simulink model "aerodynamic_model_V1_2_Wrench"  (R2025b)
settings: Solver=ode4  StartTime=0.0  StopTime=0.3  FixedStep=Ts  RelTol=1e-3
InitFcn:
  | % Run initial_main.m first to load Ad,As,Tq_prop,Tq_mass,...
values from neighbouring files (symbols this model uses):
  alpha_du0_v_tail_L = trim_aero_ic.v_tail_L.alpha_du0    [initial_main_V1_1.m]
  alpha_du0_v_tail_R = trim_aero_ic.v_tail_R.alpha_du0    [initial_main_V1_1.m]
  alpha_du0_wing_L = trim_aero_ic.wing_L.alpha_du0    [initial_main_V1_1.m]
  alpha_du0_wing_R = trim_aero_ic.wing_R.alpha_du0    [initial_main_V1_1.m]
  As = sys_sd.A    [initial_main_V1_1.m]
  BladePitch_deg = 34    [initial_main_V1_1.m]
  Bs = sys_sd.B    [initial_main_V1_1.m]
  Cs = sys_sd.C    [initial_main_V1_1.m]
  ctrl_delta_lim_deg = strips.delta_lim_deg    [initial_main_V1_1.m]
  ctrl_map_aileron_L = aero.wing_L.map_aileron(:)    [initial_main_V1_1.m]
  ctrl_map_aileron_R = aero.wing_R.map_aileron(:)    [initial_main_V1_1.m]
  ctrl_map_tail_L = aero.v_tail_L.map_tail(:)    [initial_main_V1_1.m]
  ctrl_map_tail_R = aero.v_tail_R.map_tail(:)    [initial_main_V1_1.m]
  Ds = sys_sd.D    [initial_main_V1_1.m]
  I_cg_b = R_sb * I_cg_m * R_sb.'    [aeroelastic.m]    (also in initial_main_V1_1.m = grav.I_cg_b)
  I_cg_b_inv = R_sb * I_cg_m_inv * R_sb.'    [aeroelastic.m]    (also in initial_main_V1_1.m = grav.I_cg_b_inv)
  m_node = zeros(n_id, 1)    [aeroelastic.m]    (also in generate_pullup_load_cloud.m = evalin('base', 'm_node(:)'); initial_main_V1_1.m = nodal.m_node)
  m_total_kg = evalin('base', 'm_total_kg')    [generate_pullup_load_cloud.m]    (also in initial_main_V1_1.m = grav.m_total_kg)
  n_modes = size(Phi, 2)    [aeroelastic.m]    (also in initial_main_V1_1.m = n_rigid + n_elastic)
  ones_1_tail = ones(1, size(r_cg2ac_b_v_tail_L, 2))    [initial_main_V1_1.m]
  ones_1_wing = ones(1, size(r_cg2ac_b_wing_L, 2))    [initial_main_V1_1.m]
  Phi = evalin('base', 'Phi')    [generate_pullup_load_cloud.m]    (also in initial_main_V1_1.m = strips.Phi)
  polar_alpha_deg = polar.alpha_deg(:).'    [initial_main_V1_1.m]
  polar_CD = polar.CD(:).'    [initial_main_V1_1.m]
  polar_CDp = polar.CDp(:).'    [initial_main_V1_1.m]
  polar_CL = polar.CL(:).'    [initial_main_V1_1.m]
  polar_CM = polar.CM(:).'    [initial_main_V1_1.m]
  r_cg2ac_b_v_tail_L = R_sb * aero.v_tail_L.r_ac_s    [initial_main_V1_1.m]
  r_cg2ac_b_v_tail_R = R_sb * aero.v_tail_R.r_ac_s    [initial_main_V1_1.m]
  r_cg2ac_b_wing_L = R_sb * aero.wing_L.r_ac_s    [initial_main_V1_1.m]
  r_cg2ac_b_wing_R = R_sb * aero.wing_R.r_ac_s    [initial_main_V1_1.m]
  r_cg2kink_b = eng.r_cg2kink_b    [initial_main_V1_1.m]
  r_cg2node_b = aeroelastic.node_arms(nodes, 'R_sb', R_sb).r_cg2node_b    [initial_main_V1_1.m]
  surface_nodes = aeroelastic.surface_load_nodes(nodes)    [initial_main_V1_1.m]
  T_aero2W = aeroelastic.wing_aileron_to_W(strips).T    [initial_main_V1_1.m]
  T_prop2W = load_maps.T_prop2W    [initial_main_V1_1.m]
  Tq_mass = load_maps.Tq_mass    [initial_main_V1_1.m]
  trim_Attitude_rad0 = trim_default.Attitude_rad0    [initial_main_V1_1.m]
  trim_Omega_b0 = trim_default.Omega_b0    [initial_main_V1_1.m]
  trim_Position0 = trim_default.Position0    [initial_main_V1_1.m]
  trim_Velocity_b0 = trim_default.Velocity_b0    [initial_main_V1_1.m]
  Ts = 0.001    [initial_main_V1_1.m]
  U = 55    [initial_main_V1_1.m]
  v_tail_cant_rad = deg2rad(v_tail_cant_deg)    [initial_main_V1_1.m]
  W_mass_g = grav.W_mass    [initial_main_V1_1.m]
  x0_structure = trim_default.x0_structure    [initial_main_V1_1.m]
  x0_wagner_v_tail_L = trim_aero_ic.v_tail_L.x0_wagner    [initial_main_V1_1.m]
  x0_wagner_v_tail_R = trim_aero_ic.v_tail_R.x0_wagner    [initial_main_V1_1.m]
  x0_wagner_wing_L = trim_aero_ic.wing_L.x0_wagner    [initial_main_V1_1.m]
  x0_wagner_wing_R = trim_aero_ic.wing_R.x0_wagner    [initial_main_V1_1.m]
undefined symbols (not defined in the file or in its folder): Ad_v_tail_L, Ad_v_tail_R, Ad_wing_L, Ad_wing_R, Bd_v_tail_L, Bd_v_tail_R, Bd_wing_L, Bd_wing_R, c_over_2U_v_tail_L, c_over_2U_v_tail_R, c_over_2U_wing_L, c_over_2U_wing_R, Cd_v_tail_L, Cd_v_tail_R, Cd_wing_L, Cd_wing_R, Dd_v_tail_L, Dd_v_tail_R, Dd_wing_L, Dd_wing_R, G_du_v_tail_L, G_du_v_tail_R, G_du_wing_L, G_du_wing_R, polar_aileron_alpha_deg, polar_aileron_dCD, polar_aileron_dCL, polar_aileron_dCM, polar_aileron_delta_deg, polar_ruddervator_alpha_deg, polar_ruddervator_dCD, polar_ruddervator_dCL, polar_ruddervator_dCM, polar_ruddervator_delta_deg, qS_strip_v_tail_L, qS_strip_v_tail_R, qS_strip_wing_L, qS_strip_wing_R, qSc_strip_v_tail_L, qSc_strip_v_tail_R, qSc_strip_wing_L, qSc_strip_wing_R, T_m2b_v_tail_L, T_m2b_v_tail_R, T_m2b_wing_L, T_m2b_wing_R, T_m2h_v_tail_L, T_m2h_v_tail_R, T_m2h_wing_L, T_m2h_wing_R, Tq_CM_v_tail_L, Tq_CM_v_tail_R, Tq_CM_wing_L, Tq_CM_wing_R, Tq_D_v_tail_L, Tq_D_v_tail_R, Tq_D_wing_L, Tq_D_wing_R, Tq_v_tail_L, Tq_v_tail_R ... (+2)
libraries: Prop_gryo x12, matrix_library x2
(part 5 of 6)

== system aerodynamic_model_V1_2_Wrench/Load Estimator/Engine_station1/Subsystem6 ==
  Wb_total : Inport
  r_cg_up : Inport  Port=2
  tilt_deg : Inport  Port=3
  Bus Creator : BusCreator  Inputs=6
  Bus Creator1 : BusCreator  Inputs=6
  Bus Creator2 : BusCreator  Inputs=6
  Bus Creator4 : BusCreator  Inputs=3
  Constant : Constant  Value=r_cg2node_b(:,61)
  Constant1 : Constant  Value=r_cg2node_b(:,60)
  Constant2 : Constant  Value=0
  Constant3 : Constant  Value=r_cg2node_b(:,28)
  Constant4 : Constant  Value=[0 0 0]/180*pi
  Constant5 : Constant  Value=[7 0 0]/180*pi
  Constant6 : Constant  Value=-7
  Demux{1..6} (6 alike) : Demux  Outputs=3
  Gain : Gain  Gain=pi/180
  MATLAB Function1 : MATLAB Function  TreatAsAtomicUnit=on
  MATLAB Function2 : MATLAB Function  TreatAsAtomicUnit=on
  MATLAB Function3 : MATLAB Function  TreatAsAtomicUnit=on
  Mux : Mux  Inputs=3
  Product{1..4,6..7} (6 alike) : Product  Multiplication=Matrix(*)
  Rotation Angles to Direction Cosine Matrix : Angle2Dcm  rotationOrder=XYZ
      settings: AttributesFormatString=Rotation Order: %<rotationOrder>
  Rotation Angles to Direction Cosine Matrix1 : Angle2Dcm  rotationOrder=XYZ
      settings: AttributesFormatString=Rotation Order: %<rotationOrder>
  Rotation Angles to Direction Cosine Matrix2 : Angle2Dcm  rotationOrder=XYZ
      settings: AttributesFormatString=Rotation Order: %<rotationOrder>
  Selector1 : Selector  NumberOfDimensions=2  InputPortWidth=3  IndexOptions=Select all,Index vector (dialog)  Indices=[1:6],[61]  OutputSizes=1,1
  Selector10 : Selector  NumberOfDimensions=2  InputPortWidth=3  IndexOptions=Index vector (dialog),Select all  Indices=[4:6],[surface_nodes.wing_R.node_id]  OutputSizes=1,1
  Selector11 : Selector  NumberOfDimensions=2  InputPortWidth=3  IndexOptions=Index vector (dialog),Select all  Indices=[4:6],[surface_nodes.wing_R.node_id]  OutputSizes=1,1
  Selector12 : Selector  NumberOfDimensions=2  InputPortWidth=3  IndexOptions=Index vector (dialog),Select all  Indices=[1:3],[surface_nodes.wing_R.node_id]  OutputSizes=1,1
  Selector13 : Selector  NumberOfDimensions=2  InputPortWidth=3  IndexOptions=Index vector (dialog),Select all  Indices=[4:6],[surface_nodes.wing_R.node_id]  OutputSizes=1,1
  Selector14 : Selector  NumberOfDimensions=2  InputPortWidth=3  IndexOptions=Index vector (dialog),Select all  Indices=[1:3],[surface_nodes.wing_R.node_id]  OutputSizes=1,1
  Selector2 : Selector  NumberOfDimensions=2  InputPortWidth=3  IndexOptions=Select all,Index vector (dialog)  Indices=[1:6],[60 61]  OutputSizes=1,1
  Selector3 : Selector  NumberOfDimensions=2  InputPortWidth=3  IndexOptions=Select all,Index vector (dialog)  Indices=[1:6],[61]  OutputSizes=1,1
  Selector4 : Selector  NumberOfDimensions=2  InputPortWidth=3  IndexOptions=Select all,Index vector (dialog)  Indices=[1:6],[60 61]  OutputSizes=1,1
  Selector5 : Selector  NumberOfDimensions=2  InputPortWidth=3  IndexOptions=Select all,Index vector (dialog)  Indices=[1:6],[59:61]  OutputSizes=1,1
  Selector6 : Selector  NumberOfDimensions=2  InputPortWidth=3  IndexOptions=Select all,Index vector (dialog)  Indices=[1:6],[59:61]  OutputSizes=1,1
  Selector9 : Selector  NumberOfDimensions=2  InputPortWidth=3  IndexOptions=Index vector (dialog),Select all  Indices=[1:3],[surface_nodes.wing_R.node_id]  OutputSizes=1,1
  Out1 : Outport
  wires:
  Demux3/3 -> Bus Creator2/3  "shear_forcez"
  Selector4/1 -> MATLAB Function2/3(r)
  MATLAB Function3/2(M_b) -> Product4/2
  MATLAB Function1/2(M_b) -> Product7/2
  Demux1/2 -> Bus Creator1/2  "shear_forcey"
  Demux6/3 -> Bus Creator2/6  "Bending_momenty"
  MATLAB Function1/1(F_b) -> Product6/2
  Selector6/1 -> MATLAB Function3/3(r)
  Demux1/3 -> Bus Creator1/3  "shear_forcez"
  Demux5/2 -> Bus Creator/5  "Bending_momentx"
  Selector2/1 -> Selector11/1, Selector12/1
  Demux4/2 -> Bus Creator/2  "shear_forcey"
  Selector12/1 -> MATLAB Function2/1(F)
  Bus Creator1/1 -> Bus Creator4/2
  Demux5/3 -> Bus Creator/6  "Bending_momenty"
  Selector5/1 -> Selector13/1, Selector14/1
  Constant1/1 -> MATLAB Function2/4(p)
  Demux5/1 -> Bus Creator/4  "Torision_moment"
  Constant2/1 -> Mux/3
  Gain/1 -> Rotation Angles to Direction Cosine Matrix/1
  Bus Creator2/1 -> Bus Creator4/3
  Product3/1 -> Demux3/1
  Demux1/1 -> Bus Creator1/1  "Axial_Force"
  Selector9/1 -> MATLAB Function1/1(F)
  Product7/1 -> Demux5/1
  Bus Creator/1 -> Bus Creator4/1
  Demux4/1 -> Bus Creator/1  "Axial_Force"
  Wb_total/1 -> Selector2/1, Selector5/1, Selector1/1
  Demux2/1 -> Bus Creator1/4  "Torision_moment"
  Rotation Angles to Direction Cosine Matrix2/1 -> Product4/1, Product3/1
  Constant6/1 -> Mux/1
  Mux/1 -> Gain/1
  Product6/1 -> Demux4/1
  Demux3/1 -> Bus Creator2/1  "Axial_Force"
  Selector11/1 -> MATLAB Function2/2(M)
  Demux6/1 -> Bus Creator2/4  "Torision_moment"
  Demux2/3 -> Bus Creator1/6  "Bending_momenty"
  MATLAB Function2/1(F_b) -> Product1/2
  Rotation Angles to Direction Cosine Matrix1/1 -> Product1/1, Product2/1
  Demux4/3 -> Bus Creator/3  "shear_forcez"
  Constant3/1 -> MATLAB Function3/4(p)
  Product1/1 -> Demux1/1
  Product2/1 -> Demux2/1
  Constant5/1 -> Rotation Angles to Direction Cosine Matrix1/1
  MATLAB Function2/2(M_b) -> Product2/2
  Bus Creator4/1 -> Out1/1
  r_cg_up/1 -> Selector6/1, Selector4/1, Selector3/1
  Selector1/1 -> Selector10/1, Selector9/1
  MATLAB Function3/1(F_b) -> Product3/2
  tilt_deg/1 -> Mux/2
  Selector10/1 -> MATLAB Function1/2(M)
  Rotation Angles to Direction Cosine Matrix/1 -> Product7/1, Product6/1
  Selector13/1 -> MATLAB Function3/2(M)
  Constant4/1 -> Rotation Angles to Direction Cosine Matrix2/1
  Selector14/1 -> MATLAB Function3/1(F)
  Demux2/2 -> Bus Creator1/5  "Bending_momentx"
  Demux3/2 -> Bus Creator2/2  "shear_forcey"
  Selector3/1 -> MATLAB Function1/3(r)
  Constant/1 -> MATLAB Function1/4(p)
  Demux6/2 -> Bus Creator2/5  "Bending_momentx"
  Product4/1 -> Demux6/1

== system aerodynamic_model_V1_2_Wrench/Load Estimator/Engine_station1/Subsystem7 ==
  In1 : Inport
  r_cg_up : Inport  Port=2
  Bus Creator : BusCreator  Inputs=6
  Bus Creator1 : BusCreator  Inputs=6
  Bus Creator2 : BusCreator  Inputs=6
  Bus Creator4 : BusCreator  Inputs=3
  Constant : Constant  Value=r_cg2node_b(:,67)
  Constant1 : Constant  Value=r_cg2node_b(:,66)
  Constant2 : Constant  Value=0
  Constant3 : Constant  Value=r_cg2node_b(:,46)
  Constant4 : Constant  Value=[0 0 0]/180*pi
  Constant5 : Constant  Value=[-7 0 0]/180*pi
  Constant6 : Constant  Value=-7
  Constant7 : Constant  Value=90
  Demux{1..6} (6 alike) : Demux  Outputs=3
  Gain : Gain  Gain=pi/180
  MATLAB Function1 : MATLAB Function  TreatAsAtomicUnit=on
  MATLAB Function2 : MATLAB Function  TreatAsAtomicUnit=on
  MATLAB Function3 : MATLAB Function  TreatAsAtomicUnit=on
  Mux : Mux  Inputs=3
  Product{1..4,6..7} (6 alike) : Product  Multiplication=Matrix(*)
  Rotation Angles to Direction Cosine Matrix : Angle2Dcm  rotationOrder=XYZ
      settings: AttributesFormatString=Rotation Order: %<rotationOrder>
  Rotation Angles to Direction Cosine Matrix1 : Angle2Dcm  rotationOrder=XYZ
      settings: AttributesFormatString=Rotation Order: %<rotationOrder>
  Rotation Angles to Direction Cosine Matrix2 : Angle2Dcm  rotationOrder=XYZ
      settings: AttributesFormatString=Rotation Order: %<rotationOrder>
  Selector1 : Selector  NumberOfDimensions=2  InputPortWidth=3  IndexOptions=Select all,Index vector (dialog)  Indices=[1:6],[67]  OutputSizes=1,1
  Selector10 : Selector  NumberOfDimensions=2  InputPortWidth=3  IndexOptions=Index vector (dialog),Select all  Indices=[4:6],[surface_nodes.wing_R.node_id]  OutputSizes=1,1
  Selector11 : Selector  NumberOfDimensions=2  InputPortWidth=3  IndexOptions=Index vector (dialog),Select all  Indices=[4:6],[surface_nodes.wing_R.node_id]  OutputSizes=1,1
  Selector12 : Selector  NumberOfDimensions=2  InputPortWidth=3  IndexOptions=Index vector (dialog),Select all  Indices=[1:3],[surface_nodes.wing_R.node_id]  OutputSizes=1,1
  Selector13 : Selector  NumberOfDimensions=2  InputPortWidth=3  IndexOptions=Index vector (dialog),Select all  Indices=[4:6],[surface_nodes.wing_R.node_id]  OutputSizes=1,1
  Selector14 : Selector  NumberOfDimensions=2  InputPortWidth=3  IndexOptions=Index vector (dialog),Select all  Indices=[1:3],[surface_nodes.wing_R.node_id]  OutputSizes=1,1
  Selector2 : Selector  NumberOfDimensions=2  InputPortWidth=3  IndexOptions=Select all,Index vector (dialog)  Indices=[1:6],[66 67]  OutputSizes=1,1
  Selector3 : Selector  NumberOfDimensions=2  InputPortWidth=3  IndexOptions=Select all,Index vector (dialog)  Indices=[1:6],[67]  OutputSizes=1,1
  Selector4 : Selector  NumberOfDimensions=2  InputPortWidth=3  IndexOptions=Select all,Index vector (dialog)  Indices=[1:6],[66 67]  OutputSizes=1,1
  Selector5 : Selector  NumberOfDimensions=2  InputPortWidth=3  IndexOptions=Select all,Index vector (dialog)  Indices=[1:6],[65:67]  OutputSizes=1,1
  Selector6 : Selector  NumberOfDimensions=2  InputPortWidth=3  IndexOptions=Select all,Index vector (dialog)  Indices=[1:6],[65:67]  OutputSizes=1,1
  Selector9 : Selector  NumberOfDimensions=2  InputPortWidth=3  IndexOptions=Index vector (dialog),Select all  Indices=[1:3],[surface_nodes.wing_R.node_id]  OutputSizes=1,1
  Out1 : Outport
  wires:
  Product4/1 -> Demux6/1
  Demux6/2 -> Bus Creator2/5  "Bending_momentx"
  Constant/1 -> MATLAB Function1/4(p)
  Selector3/1 -> MATLAB Function1/3(r)
  Demux3/2 -> Bus Creator2/2  "shear_forcey"
  Demux2/2 -> Bus Creator1/5  "Bending_momentx"
  Selector14/1 -> MATLAB Function3/1(F)
  Constant4/1 -> Rotation Angles to Direction Cosine Matrix2/1
  Selector13/1 -> MATLAB Function3/2(M)
  Rotation Angles to Direction Cosine Matrix/1 -> Product6/1, Product7/1
  Selector10/1 -> MATLAB Function1/2(M)
  Constant7/1 -> Mux/2
  MATLAB Function3/1(F_b) -> Product3/2
  Selector1/1 -> Selector9/1, Selector10/1
  r_cg_up/1 -> Selector3/1, Selector4/1, Selector6/1
  Bus Creator4/1 -> Out1/1
  MATLAB Function2/2(M_b) -> Product2/2
  Constant5/1 -> Rotation Angles to Direction Cosine Matrix1/1
  Product2/1 -> Demux2/1
  Product1/1 -> Demux1/1
  Constant3/1 -> MATLAB Function3/4(p)
  Demux4/3 -> Bus Creator/3  "shear_forcez"
  Rotation Angles to Direction Cosine Matrix1/1 -> Product2/1, Product1/1
  MATLAB Function2/1(F_b) -> Product1/2
  Demux2/3 -> Bus Creator1/6  "Bending_momenty"
  Demux6/1 -> Bus Creator2/4  "Torision_moment"
  Selector11/1 -> MATLAB Function2/2(M)
  Demux3/1 -> Bus Creator2/1  "Axial_Force"
  Product6/1 -> Demux4/1
  Mux/1 -> Gain/1
  Constant6/1 -> Mux/1
  Rotation Angles to Direction Cosine Matrix2/1 -> Product3/1, Product4/1
  Demux2/1 -> Bus Creator1/4  "Torision_moment"
  In1/1 -> Selector2/1, Selector5/1, Selector1/1
  Demux4/1 -> Bus Creator/1  "Axial_Force"
  Bus Creator/1 -> Bus Creator4/1
  Product7/1 -> Demux5/1
  Selector9/1 -> MATLAB Function1/1(F)
  Demux1/1 -> Bus Creator1/1  "Axial_Force"
  Product3/1 -> Demux3/1
  Bus Creator2/1 -> Bus Creator4/3
  Gain/1 -> Rotation Angles to Direction Cosine Matrix/1
  Constant2/1 -> Mux/3
  Demux5/1 -> Bus Creator/4  "Torision_moment"
  Constant1/1 -> MATLAB Function2/4(p)
  Selector5/1 -> Selector14/1, Selector13/1
  Demux5/3 -> Bus Creator/6  "Bending_momenty"
  Bus Creator1/1 -> Bus Creator4/2
  Selector12/1 -> MATLAB Function2/1(F)
  Demux4/2 -> Bus Creator/2  "shear_forcey"
  Selector2/1 -> Selector12/1, Selector11/1
  Demux5/2 -> Bus Creator/5  "Bending_momentx"
  Demux1/3 -> Bus Creator1/3  "shear_forcez"
  Selector6/1 -> MATLAB Function3/3(r)
  MATLAB Function1/1(F_b) -> Product6/2
  Demux6/3 -> Bus Creator2/6  "Bending_momenty"
  Demux1/2 -> Bus Creator1/2  "shear_forcey"
  MATLAB Function1/2(M_b) -> Product7/2
  MATLAB Function3/2(M_b) -> Product4/2
  Selector4/1 -> MATLAB Function2/3(r)
  Demux3/3 -> Bus Creator2/3  "shear_forcez"

== matlab function aerodynamic_model_V1_2_Wrench/Strip Aerodynamics/Local_Alphas/MATLAB Function1 ==
  data: V input; alpha output; beta output
function [alpha, beta] = fcn(V)
[alpha, beta] = strip_aero_angles(V);
end

== matlab function aerodynamic_model_V1_2_Wrench/Strip Aerodynamics/Local_Alphas/MATLAB Function2 ==
  data: V input; alpha output; beta output
function [alpha, beta] = fcn(V)
[alpha, beta] = strip_aero_angles(V);
end

== matlab function aerodynamic_model_V1_2_Wrench/Strip Aerodynamics/Local_Alphas/MATLAB Function4 ==
  data: V input; alpha output; beta output
function [alpha, beta] = fcn(V)
[alpha, beta] = strip_aero_angles(V);
end

== matlab function aerodynamic_model_V1_2_Wrench/Strip Aerodynamics/Local_Alphas/MATLAB Function ==
  data: omega input; Omega_skew output
function Omega_skew = fcn(omega)
p=omega(1);
q=omega(2);
r=omega(3);

Omega_skew =  [0 -r q;r 0 -p;-q p 0];

== matlab function aerodynamic_model_V1_2_Wrench/Load Estimator/Structural_Station_Section/MATLAB Function3 ==
  data: F input; F_b output; M input; r input; M_b output; p input
function [F_b, M_b] = wrench_to_cg(F, M, r,p) %#codegen
%WRENCH_TO_CG  节点力/力矩合到质心
%
%  [F_cg, M_cg] = wrench_to_cg(F, M, r)
%
%  F, M, r  3×n  每列一个节点，必须同一坐标系
%            r 用 r_cg2node_m（结构）或 r_cg2node_b（机体）
%  F_cg     3×1  Σ F
%  M_cg     3×1  Σ (r × F + M)
%
%  不要把 6 维扳手整段叉乘。力只求和；力矩才是 r×F 再加节点力矩。
n=size(r,2);
for i=1:n
    r(:,i)=r(:,i)-p;
end
    F_b = sum(F, 2);
    M_b = sum(cross3n(r, F) + M, 2);
end

== matlab function aerodynamic_model_V1_2_Wrench/Flexible Aircraft Dynamics/MATLAB Function2 ==
  data: F input; F_cg output; M input; r input; M_cg output
function [F_cg, M_cg] = wrench_to_cg(F, M, r) %#codegen
%WRENCH_TO_CG  节点力/力矩合到质心
%
%  [F_cg, M_cg] = wrench_to_cg(F, M, r)
%
%  F, M, r  3×n  每列一个节点，必须同一坐标系
%            r 用 r_cg2node_m（结构）或 r_cg2node_b（机体）
%  F_cg     3×1  Σ F
%  M_cg     3×1  Σ (r × F + M)
%
%  不要把 6 维扳手整段叉乘。力只求和；力矩才是 r×F 再加节点力矩。

    F_cg = sum(F, 2);
    M_cg = sum(cross3n(r, F) + M, 2);
end

== matlab function aerodynamic_model_V1_2_Wrench/Load Estimator/MATLAB Function2 ==
  data: V_b input; Acc_b input; a_node output; Omega_b input; rate_b input; r input; m input; F_inertia output; a_cg_up input
function [a_node, F_inertia] = rigid_node_inertia( ...
    V_b, Acc_b, Omega_b, rate_b, r, m, a_cg_up) %#codegen
%RIGID_NODE_INERTIA
% 计算刚体运动条件下各节点的绝对加速度和惯性力
%
% 输入：
%   V_b      3×1   质心速度 [u;v;w]，机体系
%   Acc_b    3×1   速度分量导数 [du/dt;dv/dt;dw/dt]
%   Omega_b  3×1   刚体角速度 [p;q;r]
%   rate_b   3×1   刚体角加速度 [dp/dt;dq/dt;dr/dt]
%   r        3×N   CG到各节点的位置矢量
%   m        N×1   各节点质量
%
% 输出：
%   a_node      3×N  各节点绝对加速度
%   F_inertia   3×N  各节点惯性力
%
% 惯性力采用达朗贝尔形式：
%
%   F_inertia_i = -m_i * a_i
%
% 要求：
%   size(r,2) == length(m)

    % 质心绝对加速度
    % 若 Acc_b 已经是绝对加速度，则这里应直接写：
    % a_cg = Acc_b;
    a_cg = Acc_b + cross(Omega_b, V_b);

    % 节点数量
    n = size(r, 2);

    % 预分配
    a_node    = a_cg_up;
    F_inertia = zeros(6, n);

    % 各节点刚体惯性载荷
    for i = 1:n

        ri = r(:,i);

        % 节点绝对加速度
        a_node(:,i) = a_node(:,i)+ a_cg ...
            + cross(rate_b, ri) ...
            + cross(Omega_b, cross(Omega_b, ri));

        % 节点惯性力
        F_inertia(1:3,i) = -m(i) * a_node(:,i);

    end

end

== matlab function aerodynamic_model_V1_2_Wrench/Flexible Aircraft Dynamics/MATLAB Function3 ==
  data: p input; phi_dot output; q input; r input; phi input; theta input; theta_dot output; psi_dot output
function [phi_dot, theta_dot, psi_dot] = euler_kinematics(p, q, r, phi, theta)
    % 输入：
    %   p, q, r  - 体轴角速度 (rad/s)
    %   phi      - 滚转角 (rad)
    %   theta    - 俯仰角 (rad)
    % 输出：
    %   phi_dot, theta_dot, psi_dot - 欧拉角变化率 (rad/s)
    
    % 保护：防止 theta = ±90° 时除零（万向节锁）
    cos_theta = cos(theta);
    if abs(cos_theta) < 1e-6
        cos_theta = sign(cos_theta) * 1e-6;  % 保留符号，避免符号跳变
    end
    
    tan_theta = sin(theta) / cos_theta;
    
    % 运动学矩阵
    phi_dot   = p + q * sin(phi) * tan_theta + r * cos(phi) * tan_theta;
    theta_dot = q * cos(phi) - r * sin(phi);
    psi_dot   = (q * sin(phi) + r * cos(phi)) / cos_theta;
end

== matlab function aerodynamic_model_V1_2_Wrench/Load Estimator/Engine_station/Subsystem/MATLAB Function1 ==
  data: F input; F_b output; M input; r input; M_b output; p input
function [F_b, M_b] = wrench_to_cg(F, M, r,p) %#codegen
%WRENCH_TO_CG  节点力/力矩合到质心
%
%  [F_cg, M_cg] = wrench_to_cg(F, M, r)
%
%  F, M, r  3×n  每列一个节点，必须同一坐标系
%            r 用 r_cg2node_m（结构）或 r_cg2node_b（机体）
%  F_cg     3×1  Σ F
%  M_cg     3×1  Σ (r × F + M)
%
%  不要把 6 维扳手整段叉乘。力只求和；力矩才是 r×F 再加节点力矩。
n=size(r,2);
for i=1:n
    r(:,i)=r(:,i)-p;
end
    F_b = sum(F, 2);
    M_b = sum(cross3n(r, F) + M, 2);
end

== matlab function aerodynamic_model_V1_2_Wrench/Load Estimator/Engine_station/Subsystem/MATLAB Function2 ==
  data: F input; F_b output; M input; r input; M_b output; p input
function [F_b, M_b] = wrench_to_cg(F, M, r,p) %#codegen
%WRENCH_TO_CG  节点力/力矩合到质心
%
%  [F_cg, M_cg] = wrench_to_cg(F, M, r)
%
%  F, M, r  3×n  每列一个节点，必须同一坐标系
%            r 用 r_cg2node_m（结构）或 r_cg2node_b（机体）
%  F_cg     3×1  Σ F
%  M_cg     3×1  Σ (r × F + M)
%
%  不要把 6 维扳手整段叉乘。力只求和；力矩才是 r×F 再加节点力矩。
n=size(r,2);
for i=1:n
    r(:,i)=r(:,i)-p;
end
    F_b = sum(F, 2);
    M_b = sum(cross3n(r, F) + M, 2);
end

== matlab function aerodynamic_model_V1_2_Wrench/Load Estimator/Engine_station/Subsystem/MATLAB Function3 ==
  data: F input; F_b output; M input; r input; M_b output; p input
function [F_b, M_b] = wrench_to_cg(F, M, r,p) %#codegen
%WRENCH_TO_CG  节点力/力矩合到质心
%
%  [F_cg, M_cg] = wrench_to_cg(F, M, r)
%
%  F, M, r  3×n  每列一个节点，必须同一坐标系
%            r 用 r_cg2node_m（结构）或 r_cg2node_b（机体）
%  F_cg     3×1  Σ F
%  M_cg     3×1  Σ (r × F + M)
%
%  不要把 6 维扳手整段叉乘。力只求和；力矩才是 r×F 再加节点力矩。
n=size(r,2);
for i=1:n
    r(:,i)=r(:,i)-p;
end
    F_b = sum(F, 2);
    M_b = sum(cross3n(r, F) + M, 2);
end

== matlab function aerodynamic_model_V1_2_Wrench/Load Estimator/Engine_station/Subsystem1/MATLAB Function1 ==
  data: F input; F_b output; M input; r input; M_b output; p input
function [F_b, M_b] = wrench_to_cg(F, M, r,p) %#codegen
%WRENCH_TO_CG  节点力/力矩合到质心
%
%  [F_cg, M_cg] = wrench_to_cg(F, M, r)
%
%  F, M, r  3×n  每列一个节点，必须同一坐标系
%            r 用 r_cg2node_m（结构）或 r_cg2node_b（机体）
%  F_cg     3×1  Σ F
%  M_cg     3×1  Σ (r × F + M)
%
%  不要把 6 维扳手整段叉乘。力只求和；力矩才是 r×F 再加节点力矩。
n=size(r,2);
for i=1:n
    r(:,i)=r(:,i)-p;
end
    F_b = sum(F, 2);
    M_b = sum(cross3n(r, F) + M, 2);
end

== matlab function aerodynamic_model_V1_2_Wrench/Load Estimator/Engine_station/Subsystem1/MATLAB Function2 ==
  data: F input; F_b output; M input; r input; M_b output; p input
function [F_b, M_b] = wrench_to_cg(F, M, r,p) %#codegen
%WRENCH_TO_CG  节点力/力矩合到质心
%
%  [F_cg, M_cg] = wrench_to_cg(F, M, r)
%
%  F, M, r  3×n  每列一个节点，必须同一坐标系
%            r 用 r_cg2node_m（结构）或 r_cg2node_b（机体）
%  F_cg     3×1  Σ F
%  M_cg     3×1  Σ (r × F + M)
%
%  不要把 6 维扳手整段叉乘。力只求和；力矩才是 r×F 再加节点力矩。
n=size(r,2);
for i=1:n
    r(:,i)=r(:,i)-p;
end
    F_b = sum(F, 2);
    M_b = sum(cross3n(r, F) + M, 2);
end

== matlab function aerodynamic_model_V1_2_Wrench/Load Estimator/Engine_station/Subsystem1/MATLAB Function3 ==
  data: F input; F_b output; M input; r input; M_b output; p input
function [F_b, M_b] = wrench_to_cg(F, M, r,p) %#codegen
%WRENCH_TO_CG  节点力/力矩合到质心
%
%  [F_cg, M_cg] = wrench_to_cg(F, M, r)
%
%  F, M, r  3×n  每列一个节点，必须同一坐标系
%            r 用 r_cg2node_m（结构）或 r_cg2node_b（机体）
%  F_cg     3×1  Σ F
%  M_cg     3×1  Σ (r × F + M)
%
%  不要把 6 维扳手整段叉乘。力只求和；力矩才是 r×F 再加节点力矩。
n=size(r,2);
for i=1:n
    r(:,i)=r(:,i)-p;
end
    F_b = sum(F, 2);
    M_b = sum(cross3n(r, F) + M, 2);
end

== matlab function aerodynamic_model_V1_2_Wrench/Load Estimator/Engine_station/Subsystem2/MATLAB Function1 ==
  data: F input; F_b output; M input; r input; M_b output; p input
function [F_b, M_b] = wrench_to_cg(F, M, r,p) %#codegen
%WRENCH_TO_CG  节点力/力矩合到质心
%
%  [F_cg, M_cg] = wrench_to_cg(F, M, r)
%
%  F, M, r  3×n  每列一个节点，必须同一坐标系
%            r 用 r_cg2node_m（结构）或 r_cg2node_b（机体）
%  F_cg     3×1  Σ F
%  M_cg     3×1  Σ (r × F + M)
%
%  不要把 6 维扳手整段叉乘。力只求和；力矩才是 r×F 再加节点力矩。
n=size(r,2);
for i=1:n
    r(:,i)=r(:,i)-p;
end
    F_b = sum(F, 2);
    M_b = sum(cross3n(r, F) + M, 2);
end

== matlab function aerodynamic_model_V1_2_Wrench/Load Estimator/Engine_station/Subsystem2/MATLAB Function2 ==
  data: F input; F_b output; M input; r input; M_b output; p input
function [F_b, M_b] = wrench_to_cg(F, M, r,p) %#codegen
%WRENCH_TO_CG  节点力/力矩合到质心
%
%  [F_cg, M_cg] = wrench_to_cg(F, M, r)
%
%  F, M, r  3×n  每列一个节点，必须同一坐标系
%            r 用 r_cg2node_m（结构）或 r_cg2node_b（机体）
%  F_cg     3×1  Σ F
%  M_cg     3×1  Σ (r × F + M)
%
%  不要把 6 维扳手整段叉乘。力只求和；力矩才是 r×F 再加节点力矩。
n=size(r,2);
for i=1:n
    r(:,i)=r(:,i)-p;
end
    F_b = sum(F, 2);
    M_b = sum(cross3n(r, F) + M, 2);
end

== matlab function aerodynamic_model_V1_2_Wrench/Load Estimator/Engine_station/Subsystem2/MATLAB Function3 ==
  data: F input; F_b output; M input; r input; M_b output; p input
function [F_b, M_b] = wrench_to_cg(F, M, r,p) %#codegen
%WRENCH_TO_CG  节点力/力矩合到质心
%
%  [F_cg, M_cg] = wrench_to_cg(F, M, r)
%
%  F, M, r  3×n  每列一个节点，必须同一坐标系
%            r 用 r_cg2node_m（结构）或 r_cg2node_b（机体）
%  F_cg     3×1  Σ F
%  M_cg     3×1  Σ (r × F + M)
%
%  不要把 6 维扳手整段叉乘。力只求和；力矩才是 r×F 再加节点力矩。
n=size(r,2);
for i=1:n
    r(:,i)=r(:,i)-p;
end
    F_b = sum(F, 2);
    M_b = sum(cross3n(r, F) + M, 2);
end

== matlab function aerodynamic_model_V1_2_Wrench/Load Estimator/Engine_station/Subsystem3/MATLAB Function1 ==
  data: F input; F_b output; M input; r input; M_b output; p input
function [F_b, M_b] = wrench_to_cg(F, M, r,p) %#codegen
%WRENCH_TO_CG  节点力/力矩合到质心
%
%  [F_cg, M_cg] = wrench_to_cg(F, M, r)
%
%  F, M, r  3×n  每列一个节点，必须同一坐标系
%            r 用 r_cg2node_m（结构）或 r_cg2node_b（机体）
%  F_cg     3×1  Σ F
%  M_cg     3×1  Σ (r × F + M)
%
%  不要把 6 维扳手整段叉乘。力只求和；力矩才是 r×F 再加节点力矩。
n=size(r,2);
for i=1:n
    r(:,i)=r(:,i)-p;
end
    F_b = sum(F, 2);
    M_b = sum(cross3n(r, F) + M, 2);
end

== matlab function aerodynamic_model_V1_2_Wrench/Load Estimator/Engine_station/Subsystem3/MATLAB Function2 ==
  data: F input; F_b output; M input; r input; M_b output; p input
function [F_b, M_b] = wrench_to_cg(F, M, r,p) %#codegen
%WRENCH_TO_CG  节点力/力矩合到质心
%
%  [F_cg, M_cg] = wrench_to_cg(F, M, r)
%
%  F, M, r  3×n  每列一个节点，必须同一坐标系
%            r 用 r_cg2node_m（结构）或 r_cg2node_b（机体）
%  F_cg     3×1  Σ F
%  M_cg     3×1  Σ (r × F + M)
%
%  不要把 6 维扳手整段叉乘。力只求和；力矩才是 r×F 再加节点力矩。
n=size(r,2);
for i=1:n
    r(:,i)=r(:,i)-p;
end
    F_b = sum(F, 2);
    M_b = sum(cross3n(r, F) + M, 2);
end

== matlab function aerodynamic_model_V1_2_Wrench/Load Estimator/Engine_station/Subsystem3/MATLAB Function3 ==
  data: F input; F_b output; M input; r input; M_b output; p input
function [F_b, M_b] = wrench_to_cg(F, M, r,p) %#codegen
%WRENCH_TO_CG  节点力/力矩合到质心
%
%  [F_cg, M_cg] = wrench_to_cg(F, M, r)
%
%  F, M, r  3×n  每列一个节点，必须同一坐标系
%            r 用 r_cg2node_m（结构）或 r_cg2node_b（机体）
%  F_cg     3×1  Σ F
%  M_cg     3×1  Σ (r × F + M)
%
%  不要把 6 维扳手整段叉乘。力只求和；力矩才是 r×F 再加节点力矩。
n=size(r,2);
for i=1:n
    r(:,i)=r(:,i)-p;
end
    F_b = sum(F, 2);
    M_b = sum(cross3n(r, F) + M, 2);
end

== matlab function aerodynamic_model_V1_2_Wrench/Load Estimator/Wing_Section/MATLAB Function1 ==
  data: F input; F_b output; M input; r input; p input; M_b output
function [F_b, M_b] = wrench_to_cg(F, M, r,p) %#codegen
%WRENCH_TO_CG  节点力/力矩合到质心
%
%  [F_cg, M_cg] = wrench_to_cg(F, M, r)
%
%  F, M, r  3×n  每列一个节点，必须同一坐标系
%            r 用 r_cg2node_m（结构）或 r_cg2node_b（机体）
%  F_cg     3×1  Σ F
%  M_cg     3×1  Σ (r × F + M)
%
%  不要把 6 维扳手整段叉乘。力只求和；力矩才是 r×F 再加节点力矩。
n=size(r,2);
for i=1:n
    r(:,i)=r(:,i)-p;
end
    F_b = sum(F, 2);
    M_b = sum(cross3n(r, F) + M, 2);
end

== matlab function aerodynamic_model_V1_2_Wrench/Load Estimator/Engine_station/Subsystem4/MATLAB Function1 ==
  data: F input; F_b output; M input; r input; M_b output; p input
function [F_b, M_b] = wrench_to_cg(F, M, r,p) %#codegen
%WRENCH_TO_CG  节点力/力矩合到质心
%
%  [F_cg, M_cg] = wrench_to_cg(F, M, r)
%
%  F, M, r  3×n  每列一个节点，必须同一坐标系
%            r 用 r_cg2node_m（结构）或 r_cg2node_b（机体）
%  F_cg     3×1  Σ F
%  M_cg     3×1  Σ (r × F + M)
%
%  不要把 6 维扳手整段叉乘。力只求和；力矩才是 r×F 再加节点力矩。
n=size(r,2);
for i=1:n
    r(:,i)=r(:,i)-p;
end
    F_b = sum(F, 2);
    M_b = sum(cross3n(r, F) + M, 2);
end

== matlab function aerodynamic_model_V1_2_Wrench/Load Estimator/Engine_station/Subsystem4/MATLAB Function2 ==
  data: F input; F_b output; M input; r input; M_b output; p input
function [F_b, M_b] = wrench_to_cg(F, M, r,p) %#codegen
%WRENCH_TO_CG  节点力/力矩合到质心
%
%  [F_cg, M_cg] = wrench_to_cg(F, M, r)
%
%  F, M, r  3×n  每列一个节点，必须同一坐标系
%            r 用 r_cg2node_m（结构）或 r_cg2node_b（机体）
%  F_cg     3×1  Σ F
%  M_cg     3×1  Σ (r × F + M)
%
%  不要把 6 维扳手整段叉乘。力只求和；力矩才是 r×F 再加节点力矩。
n=size(r,2);
for i=1:n
    r(:,i)=r(:,i)-p;
end
    F_b = sum(F, 2);
    M_b = sum(cross3n(r, F) + M, 2);
end

== matlab function aerodynamic_model_V1_2_Wrench/Load Estimator/Engine_station/Subsystem4/MATLAB Function3 ==
  data: F input; F_b output; M input; r input; M_b output; p input
function [F_b, M_b] = wrench_to_cg(F, M, r,p) %#codegen
%WRENCH_TO_CG  节点力/力矩合到质心
%
%  [F_cg, M_cg] = wrench_to_cg(F, M, r)
%
%  F, M, r  3×n  每列一个节点，必须同一坐标系
%            r 用 r_cg2node_m（结构）或 r_cg2node_b（机体）
%  F_cg     3×1  Σ F
%  M_cg     3×1  Σ (r × F + M)
%
%  不要把 6 维扳手整段叉乘。力只求和；力矩才是 r×F 再加节点力矩。
n=size(r,2);
for i=1:n
    r(:,i)=r(:,i)-p;
end
    F_b = sum(F, 2);
    M_b = sum(cross3n(r, F) + M, 2);
end

== matlab function aerodynamic_model_V1_2_Wrench/Load Estimator/Engine_station/Subsystem5/MATLAB Function1 ==
  data: F input; F_b output; M input; r input; M_b output; p input
function [F_b, M_b] = wrench_to_cg(F, M, r,p) %#codegen
%WRENCH_TO_CG  节点力/力矩合到质心
%
%  [F_cg, M_cg] = wrench_to_cg(F, M, r)
%
%  F, M, r  3×n  每列一个节点，必须同一坐标系
%            r 用 r_cg2node_m（结构）或 r_cg2node_b（机体）
%  F_cg     3×1  Σ F
%  M_cg     3×1  Σ (r × F + M)
%
%  不要把 6 维扳手整段叉乘。力只求和；力矩才是 r×F 再加节点力矩。
n=size(r,2);
for i=1:n
    r(:,i)=r(:,i)-p;
end
    F_b = sum(F, 2);
    M_b = sum(cross3n(r, F) + M, 2);
end

== matlab function aerodynamic_model_V1_2_Wrench/Load Estimator/Engine_station/Subsystem5/MATLAB Function2 ==
  data: F input; F_b output; M input; r input; M_b output; p input
function [F_b, M_b] = wrench_to_cg(F, M, r,p) %#codegen
%WRENCH_TO_CG  节点力/力矩合到质心
%
%  [F_cg, M_cg] = wrench_to_cg(F, M, r)
%
%  F, M, r  3×n  每列一个节点，必须同一坐标系
%            r 用 r_cg2node_m（结构）或 r_cg2node_b（机体）
%  F_cg     3×1  Σ F
%  M_cg     3×1  Σ (r × F + M)
%
%  不要把 6 维扳手整段叉乘。力只求和；力矩才是 r×F 再加节点力矩。
n=size(r,2);
for i=1:n
    r(:,i)=r(:,i)-p;
end
    F_b = sum(F, 2);
    M_b = sum(cross3n(r, F) + M, 2);
end

== matlab function aerodynamic_model_V1_2_Wrench/Load Estimator/Engine_station/Subsystem5/MATLAB Function3 ==
  data: F input; F_b output; M input; r input; M_b output; p input
function [F_b, M_b] = wrench_to_cg(F, M, r,p) %#codegen
%WRENCH_TO_CG  节点力/力矩合到质心
%
%  [F_cg, M_cg] = wrench_to_cg(F, M, r)
%
%  F, M, r  3×n  每列一个节点，必须同一坐标系
%            r 用 r_cg2node_m（结构）或 r_cg2node_b（机体）
%  F_cg     3×1  Σ F
%  M_cg     3×1  Σ (r × F + M)
%
%  不要把 6 维扳手整段叉乘。力只求和；力矩才是 r×F 再加节点力矩。
n=size(r,2);
for i=1:n
    r(:,i)=r(:,i)-p;
end
    F_b = sum(F, 2);
    M_b = sum(cross3n(r, F) + M, 2);
end

== matlab function aerodynamic_model_V1_2_Wrench/Load Estimator/Engine_station/Subsystem6/MATLAB Function1 ==
  data: F input; F_b output; M input; r input; M_b output; p input
function [F_b, M_b] = wrench_to_cg(F, M, r,p) %#codegen
%WRENCH_TO_CG  节点力/力矩合到质心
%
%  [F_cg, M_cg] = wrench_to_cg(F, M, r)
%
%  F, M, r  3×n  每列一个节点，必须同一坐标系
%            r 用 r_cg2node_m（结构）或 r_cg2node_b（机体）
%  F_cg     3×1  Σ F
%  M_cg     3×1  Σ (r × F + M)
%
%  不要把 6 维扳手整段叉乘。力只求和；力矩才是 r×F 再加节点力矩。
n=size(r,2);
for i=1:n
    r(:,i)=r(:,i)-p;
end
    F_b = sum(F, 2);
    M_b = sum(cross3n(r, F) + M, 2);
end

== matlab function aerodynamic_model_V1_2_Wrench/Load Estimator/Engine_station/Subsystem6/MATLAB Function2 ==
  data: F input; F_b output; M input; r input; M_b output; p input
function [F_b, M_b] = wrench_to_cg(F, M, r,p) %#codegen
%WRENCH_TO_CG  节点力/力矩合到质心
%
%  [F_cg, M_cg] = wrench_to_cg(F, M, r)
%
%  F, M, r  3×n  每列一个节点，必须同一坐标系
%            r 用 r_cg2node_m（结构）或 r_cg2node_b（机体）
%  F_cg     3×1  Σ F
%  M_cg     3×1  Σ (r × F + M)
%
%  不要把 6 维扳手整段叉乘。力只求和；力矩才是 r×F 再加节点力矩。
n=size(r,2);
for i=1:n
    r(:,i)=r(:,i)-p;
end
    F_b = sum(F, 2);
    M_b = sum(cross3n(r, F) + M, 2);
end

== matlab function aerodynamic_model_V1_2_Wrench/Load Estimator/Engine_station/Subsystem6/MATLAB Function3 ==
  data: F input; F_b output; M input; r input; M_b output; p input
function [F_b, M_b] = wrench_to_cg(F, M, r,p) %#codegen
%WRENCH_TO_CG  节点力/力矩合到质心
%
%  [F_cg, M_cg] = wrench_to_cg(F, M, r)
%
%  F, M, r  3×n  每列一个节点，必须同一坐标系
%            r 用 r_cg2node_m（结构）或 r_cg2node_b（机体）
%  F_cg     3×1  Σ F
%  M_cg     3×1  Σ (r × F + M)
%
%  不要把 6 维扳手整段叉乘。力只求和；力矩才是 r×F 再加节点力矩。
n=size(r,2);
for i=1:n
    r(:,i)=r(:,i)-p;
end
    F_b = sum(F, 2);
    M_b = sum(cross3n(r, F) + M, 2);
end

== matlab function aerodynamic_model_V1_2_Wrench/Load Estimator/Engine_station/Subsystem7/MATLAB Function1 ==
  data: F input; F_b output; M input; r input; M_b output; p input
function [F_b, M_b] = wrench_to_cg(F, M, r,p) %#codegen
%WRENCH_TO_CG  节点力/力矩合到质心
%
%  [F_cg, M_cg] = wrench_to_cg(F, M, r)
%
%  F, M, r  3×n  每列一个节点，必须同一坐标系
%            r 用 r_cg2node_m（结构）或 r_cg2node_b（机体）
%  F_cg     3×1  Σ F
%  M_cg     3×1  Σ (r × F + M)
%
%  不要把 6 维扳手整段叉乘。力只求和；力矩才是 r×F 再加节点力矩。
n=size(r,2);
for i=1:n
    r(:,i)=r(:,i)-p;
end
    F_b = sum(F, 2);
    M_b = sum(cross3n(r, F) + M, 2);
end

== matlab function aerodynamic_model_V1_2_Wrench/Load Estimator/Wing_Section/MATLAB Function2 ==
  data: F input; F_b output; M input; r input; M_b output; p input
function [F_b, M_b] = wrench_to_cg(F, M, r,p) %#codegen
%WRENCH_TO_CG  节点力/力矩合到质心
%
%  [F_cg, M_cg] = wrench_to_cg(F, M, r)
%
%  F, M, r  3×n  每列一个节点，必须同一坐标系
%            r 用 r_cg2node_m（结构）或 r_cg2node_b（机体）
%  F_cg     3×1  Σ F
%  M_cg     3×1  Σ (r × F + M)
%
%  不要把 6 维扳手整段叉乘。力只求和；力矩才是 r×F 再加节点力矩。
n=size(r,2);
for i=1:n
    r(:,i)=r(:,i)-p;
end
    F_b = sum(F, 2);
    M_b = sum(cross3n(r, F) + M, 2);
end

== matlab function aerodynamic_model_V1_2_Wrench/Load Estimator/Engine_station/Subsystem7/MATLAB Function2 ==
  data: F input; F_b output; M input; r input; M_b output; p input
function [F_b, M_b] = wrench_to_cg(F, M, r,p) %#codegen
%WRENCH_TO_CG  节点力/力矩合到质心
%
%  [F_cg, M_cg] = wrench_to_cg(F, M, r)
%
%  F, M, r  3×n  每列一个节点，必须同一坐标系
%            r 用 r_cg2node_m（结构）或 r_cg2node_b（机体）
%  F_cg     3×1  Σ F
%  M_cg     3×1  Σ (r × F + M)
%
%  不要把 6 维扳手整段叉乘。力只求和；力矩才是 r×F 再加节点力矩。
n=size(r,2);
for i=1:n
    r(:,i)=r(:,i)-p;
end
    F_b = sum(F, 2);
    M_b = sum(cross3n(r, F) + M, 2);
end

== matlab function aerodynamic_model_V1_2_Wrench/Load Estimator/Engine_station/Subsystem7/MATLAB Function3 ==
  data: F input; F_b output; M input; r input; M_b output; p input
function [F_b, M_b] = wrench_to_cg(F, M, r,p) %#codegen
%WRENCH_TO_CG  节点力/力矩合到质心
%
%  [F_cg, M_cg] = wrench_to_cg(F, M, r)
%
%  F, M, r  3×n  每列一个节点，必须同一坐标系
%            r 用 r_cg2node_m（结构）或 r_cg2node_b（机体）
%  F_cg     3×1  Σ F
%  M_cg     3×1  Σ (r × F + M)
%
%  不要把 6 维扳手整段叉乘。力只求和；力矩才是 r×F 再加节点力矩。
n=size(r,2);
for i=1:n
    r(:,i)=r(:,i)-p;
end
    F_b = sum(F, 2);
    M_b = sum(cross3n(r, F) + M, 2);
end

== matlab function aerodynamic_model_V1_2_Wrench/Load Estimator/Engine_station1/Subsystem/MATLAB Function1 ==
  data: F input; F_b output; M input; r input; M_b output; p input
function [F_b, M_b] = wrench_to_cg(F, M, r,p) %#codegen
%WRENCH_TO_CG  节点力/力矩合到质心
%
%  [F_cg, M_cg] = wrench_to_cg(F, M, r)
%
%  F, M, r  3×n  每列一个节点，必须同一坐标系
%            r 用 r_cg2node_m（结构）或 r_cg2node_b（机体）
%  F_cg     3×1  Σ F
%  M_cg     3×1  Σ (r × F + M)
%
%  不要把 6 维扳手整段叉乘。力只求和；力矩才是 r×F 再加节点力矩。
n=size(r,2);
for i=1:n
    r(:,i)=r(:,i)-p;
end
    F_b = sum(F, 2);
    M_b = sum(cross3n(r, F) + M, 2);
end

== matlab function aerodynamic_model_V1_2_Wrench/Load Estimator/Engine_station1/Subsystem/MATLAB Function2 ==
  data: F input; F_b output; M input; r input; M_b output; p input
function [F_b, M_b] = wrench_to_cg(F, M, r,p) %#codegen
%WRENCH_TO_CG  节点力/力矩合到质心
%
%  [F_cg, M_cg] = wrench_to_cg(F, M, r)
%
%  F, M, r  3×n  每列一个节点，必须同一坐标系
%            r 用 r_cg2node_m（结构）或 r_cg2node_b（机体）
%  F_cg     3×1  Σ F
%  M_cg     3×1  Σ (r × F + M)
%
%  不要把 6 维扳手整段叉乘。力只求和；力矩才是 r×F 再加节点力矩。
n=size(r,2);
for i=1:n
    r(:,i)=r(:,i)-p;
end
    F_b = sum(F, 2);
    M_b = sum(cross3n(r, F) + M, 2);
end

== matlab function aerodynamic_model_V1_2_Wrench/Load Estimator/Engine_station1/Subsystem/MATLAB Function3 ==
  data: F input; F_b output; M input; r input; M_b output; p input
function [F_b, M_b] = wrench_to_cg(F, M, r,p) %#codegen
%WRENCH_TO_CG  节点力/力矩合到质心
%
%  [F_cg, M_cg] = wrench_to_cg(F, M, r)
%
%  F, M, r  3×n  每列一个节点，必须同一坐标系
%            r 用 r_cg2node_m（结构）或 r_cg2node_b（机体）
%  F_cg     3×1  Σ F
%  M_cg     3×1  Σ (r × F + M)
%
%  不要把 6 维扳手整段叉乘。力只求和；力矩才是 r×F 再加节点力矩。
n=size(r,2);
for i=1:n
    r(:,i)=r(:,i)-p;
end
    F_b = sum(F, 2);
    M_b = sum(cross3n(r, F) + M, 2);
end

== matlab function aerodynamic_model_V1_2_Wrench/Load Estimator/Engine_station1/Subsystem1/MATLAB Function1 ==
  data: F input; F_b output; M input; r input; M_b output; p input
function [F_b, M_b] = wrench_to_cg(F, M, r,p) %#codegen
%WRENCH_TO_CG  节点力/力矩合到质心
%
%  [F_cg, M_cg] = wrench_to_cg(F, M, r)
%
%  F, M, r  3×n  每列一个节点，必须同一坐标系
%            r 用 r_cg2node_m（结构）或 r_cg2node_b（机体）
%  F_cg     3×1  Σ F
%  M_cg     3×1  Σ (r × F + M)
%
%  不要把 6 维扳手整段叉乘。力只求和；力矩才是 r×F 再加节点力矩。
n=size(r,2);
for i=1:n
    r(:,i)=r(:,i)-p;
end
    F_b = sum(F, 2);
    M_b = sum(cross3n(r, F) + M, 2);
end

== matlab function aerodynamic_model_V1_2_Wrench/Load Estimator/Engine_station1/Subsystem1/MATLAB Function2 ==
  data: F input; F_b output; M input; r input; M_b output; p input
function [F_b, M_b] = wrench_to_cg(F, M, r,p) %#codegen
%WRENCH_TO_CG  节点力/力矩合到质心
%
%  [F_cg, M_cg] = wrench_to_cg(F, M, r)
%
%  F, M, r  3×n  每列一个节点，必须同一坐标系
%            r 用 r_cg2node_m（结构）或 r_cg2node_b（机体）
%  F_cg     3×1  Σ F
%  M_cg     3×1  Σ (r × F + M)
%
%  不要把 6 维扳手整段叉乘。力只求和；力矩才是 r×F 再加节点力矩。
n=size(r,2);
for i=1:n
    r(:,i)=r(:,i)-p;
end
    F_b = sum(F, 2);
    M_b = sum(cross3n(r, F) + M, 2);
end

== matlab function aerodynamic_model_V1_2_Wrench/Load Estimator/Engine_station1/Subsystem1/MATLAB Function3 ==
  data: F input; F_b output; M input; r input; M_b output; p input
function [F_b, M_b] = wrench_to_cg(F, M, r,p) %#codegen
%WRENCH_TO_CG  节点力/力矩合到质心
%
%  [F_cg, M_cg] = wrench_to_cg(F, M, r)
%
%  F, M, r  3×n  每列一个节点，必须同一坐标系
%            r 用 r_cg2node_m（结构）或 r_cg2node_b（机体）
%  F_cg     3×1  Σ F
%  M_cg     3×1  Σ (r × F + M)
%
%  不要把 6 维扳手整段叉乘。力只求和；力矩才是 r×F 再加节点力矩。
n=size(r,2);
for i=1:n
    r(:,i)=r(:,i)-p;
end
    F_b = sum(F, 2);
    M_b = sum(cross3n(r, F) + M, 2);
end

== matlab function aerodynamic_model_V1_2_Wrench/Load Estimator/Engine_station1/Subsystem2/MATLAB Function1 ==
  data: F input; F_b output; M input; r input; M_b output; p input
function [F_b, M_b] = wrench_to_cg(F, M, r,p) %#codegen
%WRENCH_TO_CG  节点力/力矩合到质心
%
%  [F_cg, M_cg] = wrench_to_cg(F, M, r)
%
%  F, M, r  3×n  每列一个节点，必须同一坐标系
%            r 用 r_cg2node_m（结构）或 r_cg2node_b（机体）
%  F_cg     3×1  Σ F
%  M_cg     3×1  Σ (r × F + M)
%
%  不要把 6 维扳手整段叉乘。力只求和；力矩才是 r×F 再加节点力矩。
n=size(r,2);
for i=1:n
    r(:,i)=r(:,i)-p;
end
    F_b = sum(F, 2);
    M_b = sum(cross3n(r, F) + M, 2);
end

== matlab function aerodynamic_model_V1_2_Wrench/Load Estimator/Engine_station1/Subsystem2/MATLAB Function2 ==
  data: F input; F_b output; M input; r input; M_b output; p input
function [F_b, M_b] = wrench_to_cg(F, M, r,p) %#codegen
%WRENCH_TO_CG  节点力/力矩合到质心
%
%  [F_cg, M_cg] = wrench_to_cg(F, M, r)
%
%  F, M, r  3×n  每列一个节点，必须同一坐标系
%            r 用 r_cg2node_m（结构）或 r_cg2node_b（机体）
%  F_cg     3×1  Σ F
%  M_cg     3×1  Σ (r × F + M)
%
%  不要把 6 维扳手整段叉乘。力只求和；力矩才是 r×F 再加节点力矩。
n=size(r,2);
for i=1:n
    r(:,i)=r(:,i)-p;
end
    F_b = sum(F, 2);
    M_b = sum(cross3n(r, F) + M, 2);
end

== matlab function aerodynamic_model_V1_2_Wrench/Load Estimator/Wing_Section/MATLAB Function3 ==
  data: F input; F_b output; M input; r input; M_b output; p input
function [F_b, M_b] = wrench_to_cg(F, M, r,p) %#codegen
%WRENCH_TO_CG  节点力/力矩合到质心
%
%  [F_cg, M_cg] = wrench_to_cg(F, M, r)
%
%  F, M, r  3×n  每列一个节点，必须同一坐标系
%            r 用 r_cg2node_m（结构）或 r_cg2node_b（机体）
%  F_cg     3×1  Σ F
%  M_cg     3×1  Σ (r × F + M)
%
%  不要把 6 维扳手整段叉乘。力只求和；力矩才是 r×F 再加节点力矩。
n=size(r,2);
for i=1:n
    r(:,i)=r(:,i)-p;
end
    F_b = sum(F, 2);
    M_b = sum(cross3n(r, F) + M, 2);
end

== matlab function aerodynamic_model_V1_2_Wrench/Load Estimator/Engine_station1/Subsystem2/MATLAB Function3 ==
  data: F input; F_b output; M input; r input; M_b output; p input
function [F_b, M_b] = wrench_to_cg(F, M, r,p) %#codegen
%WRENCH_TO_CG  节点力/力矩合到质心
%
%  [F_cg, M_cg] = wrench_to_cg(F, M, r)
%
%  F, M, r  3×n  每列一个节点，必须同一坐标系
%            r 用 r_cg2node_m（结构）或 r_cg2node_b（机体）
%  F_cg     3×1  Σ F
%  M_cg     3×1  Σ (r × F + M)
%
%  不要把 6 维扳手整段叉乘。力只求和；力矩才是 r×F 再加节点力矩。
n=size(r,2);
for i=1:n
    r(:,i)=r(:,i)-p;
end
    F_b = sum(F, 2);
    M_b = sum(cross3n(r, F) + M, 2);
end

== matlab function aerodynamic_model_V1_2_Wrench/Load Estimator/Engine_station1/Subsystem3/MATLAB Function1 ==
  data: F input; F_b output; M input; r input; M_b output; p input
function [F_b, M_b] = wrench_to_cg(F, M, r,p) %#codegen
%WRENCH_TO_CG  节点力/力矩合到质心
%
%  [F_cg, M_cg] = wrench_to_cg(F, M, r)
%
%  F, M, r  3×n  每列一个节点，必须同一坐标系
%            r 用 r_cg2node_m（结构）或 r_cg2node_b（机体）
%  F_cg     3×1  Σ F
%  M_cg     3×1  Σ (r × F + M)
%
%  不要把 6 维扳手整段叉乘。力只求和；力矩才是 r×F 再加节点力矩。
n=size(r,2);
for i=1:n
    r(:,i)=r(:,i)-p;
end
    F_b = sum(F, 2);
    M_b = sum(cross3n(r, F) + M, 2);
end

== matlab function aerodynamic_model_V1_2_Wrench/Load Estimator/Engine_station1/Subsystem3/MATLAB Function2 ==
  data: F input; F_b output; M input; r input; M_b output; p input
function [F_b, M_b] = wrench_to_cg(F, M, r,p) %#codegen
%WRENCH_TO_CG  节点力/力矩合到质心
%
%  [F_cg, M_cg] = wrench_to_cg(F, M, r)
%
%  F, M, r  3×n  每列一个节点，必须同一坐标系
%            r 用 r_cg2node_m（结构）或 r_cg2node_b（机体）
%  F_cg     3×1  Σ F
%  M_cg     3×1  Σ (r × F + M)
%
%  不要把 6 维扳手整段叉乘。力只求和；力矩才是 r×F 再加节点力矩。
n=size(r,2);
for i=1:n
    r(:,i)=r(:,i)-p;
end
    F_b = sum(F, 2);
    M_b = sum(cross3n(r, F) + M, 2);
end

== matlab function aerodynamic_model_V1_2_Wrench/Load Estimator/Engine_station1/Subsystem3/MATLAB Function3 ==
  data: F input; F_b output; M input; r input; M_b output; p input
function [F_b, M_b] = wrench_to_cg(F, M, r,p) %#codegen
%WRENCH_TO_CG  节点力/力矩合到质心
%
%  [F_cg, M_cg] = wrench_to_cg(F, M, r)
%
%  F, M, r  3×n  每列一个节点，必须同一坐标系
%            r 用 r_cg2node_m（结构）或 r_cg2node_b（机体）
%  F_cg     3×1  Σ F
%  M_cg     3×1  Σ (r × F + M)
%
%  不要把 6 维扳手整段叉乘。力只求和；力矩才是 r×F 再加节点力矩。
n=size(r,2);
for i=1:n
    r(:,i)=r(:,i)-p;
end
    F_b = sum(F, 2);
    M_b = sum(cross3n(r, F) + M, 2);
end

== matlab function aerodynamic_model_V1_2_Wrench/Load Estimator/Engine_station1/Subsystem4/MATLAB Function1 ==
  data: F input; F_b output; M input; r input; M_b output; p input
function [F_b, M_b] = wrench_to_cg(F, M, r,p) %#codegen
%WRENCH_TO_CG  节点力/力矩合到质心
%
%  [F_cg, M_cg] = wrench_to_cg(F, M, r)
%
%  F, M, r  3×n  每列一个节点，必须同一坐标系
%            r 用 r_cg2node_m（结构）或 r_cg2node_b（机体）
%  F_cg     3×1  Σ F
%  M_cg     3×1  Σ (r × F + M)
%
%  不要把 6 维扳手整段叉乘。力只求和；力矩才是 r×F 再加节点力矩。
n=size(r,2);
for i=1:n
    r(:,i)=r(:,i)-p;
end
    F_b = sum(F, 2);
    M_b = sum(cross3n(r, F) + M, 2);
end

== matlab function aerodynamic_model_V1_2_Wrench/Load Estimator/Engine_station1/Subsystem4/MATLAB Function2 ==
  data: F input; F_b output; M input; r input; M_b output; p input
function [F_b, M_b] = wrench_to_cg(F, M, r,p) %#codegen
%WRENCH_TO_CG  节点力/力矩合到质心
%
%  [F_cg, M_cg] = wrench_to_cg(F, M, r)
%
%  F, M, r  3×n  每列一个节点，必须同一坐标系
%            r 用 r_cg2node_m（结构）或 r_cg2node_b（机体）
%  F_cg     3×1  Σ F
%  M_cg     3×1  Σ (r × F + M)
%
%  不要把 6 维扳手整段叉乘。力只求和；力矩才是 r×F 再加节点力矩。
n=size(r,2);
for i=1:n
    r(:,i)=r(:,i)-p;
end
    F_b = sum(F, 2);
    M_b = sum(cross3n(r, F) + M, 2);
end

== matlab function aerodynamic_model_V1_2_Wrench/Load Estimator/Engine_station1/Subsystem4/MATLAB Function3 ==
  data: F input; F_b output; M input; r input; M_b output; p input
function [F_b, M_b] = wrench_to_cg(F, M, r,p) %#codegen
%WRENCH_TO_CG  节点力/力矩合到质心
%
%  [F_cg, M_cg] = wrench_to_cg(F, M, r)
%
%  F, M, r  3×n  每列一个节点，必须同一坐标系
%            r 用 r_cg2node_m（结构）或 r_cg2node_b（机体）
%  F_cg     3×1  Σ F
%  M_cg     3×1  Σ (r × F + M)
%
%  不要把 6 维扳手整段叉乘。力只求和；力矩才是 r×F 再加节点力矩。
n=size(r,2);
for i=1:n
    r(:,i)=r(:,i)-p;
end
    F_b = sum(F, 2);
    M_b = sum(cross3n(r, F) + M, 2);
end

== matlab function aerodynamic_model_V1_2_Wrench/Load Estimator/Engine_station1/Subsystem5/MATLAB Function1 ==
  data: F input; F_b output; M input; r input; M_b output; p input
function [F_b, M_b] = wrench_to_cg(F, M, r,p) %#codegen
%WRENCH_TO_CG  节点力/力矩合到质心
%
%  [F_cg, M_cg] = wrench_to_cg(F, M, r)
%
%  F, M, r  3×n  每列一个节点，必须同一坐标系
%            r 用 r_cg2node_m（结构）或 r_cg2node_b（机体）
%  F_cg     3×1  Σ F
%  M_cg     3×1  Σ (r × F + M)
%
%  不要把 6 维扳手整段叉乘。力只求和；力矩才是 r×F 再加节点力矩。
n=size(r,2);
for i=1:n
    r(:,i)=r(:,i)-p;
end
    F_b = sum(F, 2);
    M_b = sum(cross3n(r, F) + M, 2);
end

== matlab function aerodynamic_model_V1_2_Wrench/Load Estimator/Engine_station1/Subsystem5/MATLAB Function2 ==
  data: F input; F_b output; M input; r input; M_b output; p input
function [F_b, M_b] = wrench_to_cg(F, M, r,p) %#codegen
%WRENCH_TO_CG  节点力/力矩合到质心
%
%  [F_cg, M_cg] = wrench_to_cg(F, M, r)
%
%  F, M, r  3×n  每列一个节点，必须同一坐标系
%            r 用 r_cg2node_m（结构）或 r_cg2node_b（机体）
%  F_cg     3×1  Σ F
%  M_cg     3×1  Σ (r × F + M)
%
%  不要把 6 维扳手整段叉乘。力只求和；力矩才是 r×F 再加节点力矩。
n=size(r,2);
for i=1:n
    r(:,i)=r(:,i)-p;
end
    F_b = sum(F, 2);
    M_b = sum(cross3n(r, F) + M, 2);
end

== matlab function aerodynamic_model_V1_2_Wrench/Load Estimator/Engine_station1/Subsystem5/MATLAB Function3 ==
  data: F input; F_b output; M input; r input; M_b output; p input
function [F_b, M_b] = wrench_to_cg(F, M, r,p) %#codegen
%WRENCH_TO_CG  节点力/力矩合到质心
%
%  [F_cg, M_cg] = wrench_to_cg(F, M, r)
%
%  F, M, r  3×n  每列一个节点，必须同一坐标系
%            r 用 r_cg2node_m（结构）或 r_cg2node_b（机体）
%  F_cg     3×1  Σ F
%  M_cg     3×1  Σ (r × F + M)
%
%  不要把 6 维扳手整段叉乘。力只求和；力矩才是 r×F 再加节点力矩。
n=size(r,2);
for i=1:n
    r(:,i)=r(:,i)-p;
end
    F_b = sum(F, 2);
    M_b = sum(cross3n(r, F) + M, 2);
end

== matlab function aerodynamic_model_V1_2_Wrench/Load Estimator/Wing_Section/MATLAB Function4 ==
  data: F input; F_b output; M input; r input; M_b output; p input
function [F_b, M_b] = wrench_to_cg(F, M, r,p) %#codegen
%WRENCH_TO_CG  节点力/力矩合到质心
%
%  [F_cg, M_cg] = wrench_to_cg(F, M, r)
%
%  F, M, r  3×n  每列一个节点，必须同一坐标系
%            r 用 r_cg2node_m（结构）或 r_cg2node_b（机体）
%  F_cg     3×1  Σ F
%  M_cg     3×1  Σ (r × F + M)
%
%  不要把 6 维扳手整段叉乘。力只求和；力矩才是 r×F 再加节点力矩。
n=size(r,2);
for i=1:n
    r(:,i)=r(:,i)-p;
end
    F_b = sum(F, 2);
    M_b = sum(cross3n(r, F) + M, 2);
end

== matlab function aerodynamic_model_V1_2_Wrench/Load Estimator/Engine_station1/Subsystem6/MATLAB Function1 ==
  data: F input; F_b output; M input; r input; M_b output; p input
function [F_b, M_b] = wrench_to_cg(F, M, r,p) %#codegen
%WRENCH_TO_CG  节点力/力矩合到质心
%
%  [F_cg, M_cg] = wrench_to_cg(F, M, r)
%
%  F, M, r  3×n  每列一个节点，必须同一坐标系
%            r 用 r_cg2node_m（结构）或 r_cg2node_b（机体）
%  F_cg     3×1  Σ F
%  M_cg     3×1  Σ (r × F + M)
%
%  不要把 6 维扳手整段叉乘。力只求和；力矩才是 r×F 再加节点力矩。
n=size(r,2);
for i=1:n
    r(:,i)=r(:,i)-p;
end
    F_b = sum(F, 2);
    M_b = sum(cross3n(r, F) + M, 2);
end

== matlab function aerodynamic_model_V1_2_Wrench/Load Estimator/Engine_station1/Subsystem6/MATLAB Function2 ==
  data: F input; F_b output; M input; r input; M_b output; p input
function [F_b, M_b] = wrench_to_cg(F, M, r,p) %#codegen
%WRENCH_TO_CG  节点力/力矩合到质心
%
%  [F_cg, M_cg] = wrench_to_cg(F, M, r)
%
%  F, M, r  3×n  每列一个节点，必须同一坐标系
%            r 用 r_cg2node_m（结构）或 r_cg2node_b（机体）
%  F_cg     3×1  Σ F
%  M_cg     3×1  Σ (r × F + M)
%
%  不要把 6 维扳手整段叉乘。力只求和；力矩才是 r×F 再加节点力矩。
n=size(r,2);
for i=1:n
    r(:,i)=r(:,i)-p;
end
    F_b = sum(F, 2);
    M_b = sum(cross3n(r, F) + M, 2);
end

== matlab function aerodynamic_model_V1_2_Wrench/Load Estimator/Engine_station1/Subsystem6/MATLAB Function3 ==
  data: F input; F_b output; M input; r input; M_b output; p input
function [F_b, M_b] = wrench_to_cg(F, M, r,p) %#codegen
%WRENCH_TO_CG  节点力/力矩合到质心
%
%  [F_cg, M_cg] = wrench_to_cg(F, M, r)
%
%  F, M, r  3×n  每列一个节点，必须同一坐标系
%            r 用 r_cg2node_m（结构）或 r_cg2node_b（机体）
%  F_cg     3×1  Σ F
%  M_cg     3×1  Σ (r × F + M)
%
%  不要把 6 维扳手整段叉乘。力只求和；力矩才是 r×F 再加节点力矩。
n=size(r,2);
for i=1:n
    r(:,i)=r(:,i)-p;
end
    F_b = sum(F, 2);
    M_b = sum(cross3n(r, F) + M, 2);
end
